simulink model "HFMA_4B_1_5_9_13"  (R2026b)
settings: Solver=FixedStepDiscrete  StopTime=stopTime  FixedStep=Ts
PreLoadFcn:
  | load('a_luts.mat')
values from neighbouring files (symbols this model uses):
  cosLUT = [1 1 1 1 1 1 1 1 1 1 1 1 ... (640 elements, 16x40)]    [iq_luts.mat]
  k_avg = 10    [Simulink_DOA_Test.m]    (also in collect_ranges.m; optimised_error_code.m)
  sinLUT = [0 0 0 0 0 0 0 0 0 0 0 0 ... (640 elements, 16x40)]    [iq_luts.mat]
  Ts = 1/8000    (= 0.000125)    [Simulink_DOA_Test.m]    (also in collect_ranges.m; optimised_error_code.m)
undefined symbols (not defined in the file or in its folder): a2_Im, a2_Re, a3_Im, a3_Re, NumBits1, NumBits2, Slope1, Slope2
libraries: hdlsllib x4, sl_signal_attributes x2
(part 5 of 6)

== system HFMA_4B_1_5_9_13/Subsystem/HFMA9/I//Q Separation2 ==
  note: -2x[n]*sin((2*pi*f0*n)/fs)
  note: 2x[n]*cos((2*pi*f0*n)/fs)
  Microphone Input : Inport
  F0 Index : Inport  Port=2
  IQ Counter Input : Inport  Port=3
  Gain : Gain  Gain=-2  ParamDataTypeStr=fixdt(1,18,16)  OutDataTypeStr=fixdt(1,18,14)  SaturateOnIntegerOverflow=on
  Gain1 : Gain  Gain=2  ParamDataTypeStr=fixdt(0,18,16)  OutDataTypeStr=fixdt(1,18,14)  SaturateOnIntegerOverflow=on
  IdxConv{,1..3} (4 alike) : DataTypeConversion  OutDataTypeStr=uint8  RndMeth=Floor
  Product : Product  OutDataTypeStr=fixdt(1,18,15)  SaturateOnIntegerOverflow=on
  Product1 : Product  OutDataTypeStr=fixdt(1,18,15)  SaturateOnIntegerOverflow=on
  cosLUT : LookupNDDirect  Table=[cosLUT]  TableDataTypeStr=fixdt(1,18,16)
  sinLUT : LookupNDDirect  Table=[sinLUT]  TableDataTypeStr=fixdt(1,18,16)
  I[n] : Outport
  Q[n] : Outport  Port=2
  wires:
  Gain/1 -> Q[n]/1
  Gain1/1 -> I[n]/1
  Microphone Input/1 -> Product1/1, Product/1
  cosLUT/1 -> Product/2
  sinLUT/1 -> Product1/2
  Product/1 -> Gain1/1
  Product1/1 -> Gain/1
  F0 Index/1 -> IdxConv/1, IdxConv2/1
  IQ Counter Input/1 -> IdxConv1/1, IdxConv3/1
  IdxConv/1 -> cosLUT/1
  IdxConv1/1 -> cosLUT/2
  IdxConv2/1 -> sinLUT/1
  IdxConv3/1 -> sinLUT/2

== system HFMA_4B_1_5_9_13/Subsystem/HFMA9/I//Q Separation3 ==
  note: -2x[n]*sin((2*pi*f0*n)/fs)
  note: 2x[n]*cos((2*pi*f0*n)/fs)
  Microphone Input : Inport
  F0 Index : Inport  Port=2
  IQ Counter Input : Inport  Port=3
  Gain : Gain  Gain=-2  ParamDataTypeStr=fixdt(1,18,16)  OutDataTypeStr=fixdt(1,18,14)  SaturateOnIntegerOverflow=on
  Gain1 : Gain  Gain=2  ParamDataTypeStr=fixdt(0,18,16)  OutDataTypeStr=fixdt(1,18,14)  SaturateOnIntegerOverflow=on
  IdxConv{,1..3} (4 alike) : DataTypeConversion  OutDataTypeStr=uint8  RndMeth=Floor
  Product : Product  OutDataTypeStr=fixdt(1,18,15)  SaturateOnIntegerOverflow=on
  Product1 : Product  OutDataTypeStr=fixdt(1,18,15)  SaturateOnIntegerOverflow=on
  cosLUT : LookupNDDirect  Table=[cosLUT]  TableDataTypeStr=fixdt(1,18,16)
  sinLUT : LookupNDDirect  Table=[sinLUT]  TableDataTypeStr=fixdt(1,18,16)
  I[n] : Outport
  Q[n] : Outport  Port=2
  wires:
  Gain/1 -> Q[n]/1
  Gain1/1 -> I[n]/1
  Microphone Input/1 -> Product1/1, Product/1
  cosLUT/1 -> Product/2
  sinLUT/1 -> Product1/2
  Product/1 -> Gain1/1
  Product1/1 -> Gain/1
  F0 Index/1 -> IdxConv/1, IdxConv2/1
  IQ Counter Input/1 -> IdxConv1/1, IdxConv3/1
  IdxConv/1 -> cosLUT/1
  IdxConv1/1 -> cosLUT/2
  IdxConv2/1 -> sinLUT/1
  IdxConv3/1 -> sinLUT/2

== system HFMA_4B_1_5_9_13/Subsystem/Max Theta Selector/Compare To Constant ==
  u : Inport
  Compare : RelationalOperator  Operator=<=  OutDataTypeStr=boolean
  Constant : Constant  DisableCoverage=on  Value=const  OutDataTypeStr=Inherit: Inherit via back propagation  SampleTime=-1
  y : Outport
  wires:
  Compare/1 -> y/1
  Constant/1 -> Compare/2
  u/1 -> Compare/1

== system HFMA_4B_1_5_9_13/Subsystem/Max Theta Selector/Compare To Constant1 ==
  u : Inport
  Compare : RelationalOperator  Operator===  OutDataTypeStr=boolean
  Constant : Constant  DisableCoverage=on  Value=const  OutDataTypeStr=Inherit: Inherit via back propagation  SampleTime=-1
  y : Outport
  wires:
  Compare/1 -> y/1
  Constant/1 -> Compare/2
  u/1 -> Compare/1

== system HFMA_4B_1_5_9_13/Subsystem/HFMA1/Covariance Matrix/R1 ==
  Xi_Re : Inport
  Xi_Im : Inport  Port=2
  Xj_Re : Inport  Port=3
  Xj_Im : Inport  Port=4
  RESET : Inport  Port=5
  Leaky Average : Subsystem
  Leaky Average1 : Subsystem
  ac_bd : Subsystem
  bc_ad : Subsystem
  Rij_Re : Outport
  Rij_Im : Outport  Port=2
  wires:
  Xi_Im/1 -> bc_ad/2(In2), ac_bd/2(In2)
  Xj_Im/1 -> bc_ad/4(In4), ac_bd/4(In4)
  Xj_Re/1 -> bc_ad/3(In3), ac_bd/3(In3)
  Xi_Re/1 -> bc_ad/1(In1), ac_bd/1(In1)
  ac_bd/1(Out1) -> Leaky Average/1(p[n])
  bc_ad/1(Out1) -> Leaky Average1/1(p[n])
  Leaky Average/1(Rij Out) -> Rij_Re/1
  RESET/1 -> Leaky Average1/2(RESET), Leaky Average/2(RESET)
  Leaky Average1/1(Rij Out) -> Rij_Im/1

== system HFMA_4B_1_5_9_13/Subsystem/HFMA1/Covariance Matrix/R2 ==
  Xi_Re : Inport
  Xi_Im : Inport  Port=2
  Xj_Re : Inport  Port=3
  Xj_Im : Inport  Port=4
  RESET : Inport  Port=5
  Leaky Average : Subsystem
  Leaky Average1 : Subsystem
  ac_bd : Subsystem
  bc_ad : Subsystem
  Rij_Re : Outport
  Rij_Im : Outport  Port=2
  wires:
  Xi_Im/1 -> bc_ad/2(In2), ac_bd/2(In2)
  Xj_Im/1 -> bc_ad/4(In4), ac_bd/4(In4)
  Xj_Re/1 -> bc_ad/3(In3), ac_bd/3(In3)
  Xi_Re/1 -> bc_ad/1(In1), ac_bd/1(In1)
  ac_bd/1(Out1) -> Leaky Average/1(p[n])
  bc_ad/1(Out1) -> Leaky Average1/1(p[n])
  Leaky Average/1(Rij Out) -> Rij_Re/1
  RESET/1 -> Leaky Average1/2(RESET), Leaky Average/2(RESET)
  Leaky Average1/1(Rij Out) -> Rij_Im/1

== system HFMA_4B_1_5_9_13/Subsystem/HFMA1/Covariance Matrix/R21 ==
  Xi_Re : Inport
  Xi_Im : Inport  Port=2
  Xj_Re : Inport  Port=3
  Xj_Im : Inport  Port=4
  RESET : Inport  Port=5
  Leaky Average : Subsystem
  Leaky Average1 : Subsystem
  ac_bd : Subsystem
  bc_ad : Subsystem
  Rij_Re : Outport
  Rij_Im : Outport  Port=2
  wires:
  Xi_Im/1 -> bc_ad/2(In2), ac_bd/2(In2)
  Xj_Im/1 -> bc_ad/4(In4), ac_bd/4(In4)
  Xj_Re/1 -> bc_ad/3(In3), ac_bd/3(In3)
  Xi_Re/1 -> bc_ad/1(In1), ac_bd/1(In1)
  ac_bd/1(Out1) -> Leaky Average/1(p[n])
  bc_ad/1(Out1) -> Leaky Average1/1(p[n])
  Leaky Average/1(Rij Out) -> Rij_Re/1
  RESET/1 -> Leaky Average1/2(RESET), Leaky Average/2(RESET)
  Leaky Average1/1(Rij Out) -> Rij_Im/1

== system HFMA_4B_1_5_9_13/Subsystem/HFMA1/Hardware Friendly MUSIC Algorithm/complex multiplier1 ==
  note: Rij'*an = (xu - yv) + j(xv+yu)
  x : Inport
  y : Inport  Port=2
  u : Inport  Port=3
  v : Inport  Port=4
  Add : Sum  Inputs=+-  OutDataTypeStr=fixdt(1,32,29)  SaturateOnIntegerOverflow=on
  Add1 : Sum  OutDataTypeStr=fixdt(1,32,29)  SaturateOnIntegerOverflow=on
  Product{,1..3} (4 alike) : Product  OutDataTypeStr=fixdt(1,32,29)  SaturateOnIntegerOverflow=on
  Re : Outport
  Im : Outport  Port=2
  wires:
  x/1 -> Product2/1, Product/1
  u/1 -> Product3/2, Product/2
  y/1 -> Product3/1, Product1/1
  v/1 -> Product2/2, Product1/2
  Product/1 -> Add/1
  Product1/1 -> Add/2
  Product2/1 -> Add1/1
  Product3/1 -> Add1/2
  Add/1 -> Re/1
  Add1/1 -> Im/1

== system HFMA_4B_1_5_9_13/Subsystem/HFMA1/Hardware Friendly MUSIC Algorithm/complex multiplier2 ==
  note: Rij'*an = (xu - yv) + j(xv+yu)
  x : Inport
  y : Inport  Port=2
  u : Inport  Port=3
  v : Inport  Port=4
  Add : Sum  Inputs=+-  OutDataTypeStr=fixdt(1,32,29)  SaturateOnIntegerOverflow=on
  Add1 : Sum  OutDataTypeStr=fixdt(1,32,29)  SaturateOnIntegerOverflow=on
  Product{,1..3} (4 alike) : Product  OutDataTypeStr=fixdt(1,32,29)  SaturateOnIntegerOverflow=on
  Re : Outport
  Im : Outport  Port=2
  wires:
  x/1 -> Product2/1, Product/1
  u/1 -> Product3/2, Product/2
  y/1 -> Product3/1, Product1/1
  v/1 -> Product2/2, Product1/2
  Product/1 -> Add/1
  Product1/1 -> Add/2
  Product2/1 -> Add1/1
  Product3/1 -> Add1/2
  Add/1 -> Re/1
  Add1/1 -> Im/1

== system HFMA_4B_1_5_9_13/Subsystem/HFMA1/Hardware Friendly MUSIC Algorithm/complex multiplier3 ==
  note: Rij'*an = (xu - yv) + j(xv+yu)
  x : Inport
  y : Inport  Port=2
  u : Inport  Port=3
  v : Inport  Port=4
  Add : Sum  Inputs=+-  OutDataTypeStr=fixdt(1,32,29)  SaturateOnIntegerOverflow=on
  Add1 : Sum  OutDataTypeStr=fixdt(1,32,29)  SaturateOnIntegerOverflow=on
  Product{,1..3} (4 alike) : Product  OutDataTypeStr=fixdt(1,32,29)  SaturateOnIntegerOverflow=on
  Re : Outport
  Im : Outport  Port=2
  wires:
  x/1 -> Product2/1, Product/1
  u/1 -> Product3/2, Product/2
  y/1 -> Product3/1, Product1/1
  v/1 -> Product2/2, Product1/2
  Product/1 -> Add/1
  Product1/1 -> Add/2
  Product2/1 -> Add1/1
  Product3/1 -> Add1/2
  Add/1 -> Re/1
  Add1/1 -> Im/1

== system HFMA_4B_1_5_9_13/Subsystem/HFMA13/Covariance Matrix/R1 ==
  Xi_Re : Inport
  Xi_Im : Inport  Port=2
  Xj_Re : Inport  Port=3
  Xj_Im : Inport  Port=4
  RESET : Inport  Port=5
  Leaky Average : Subsystem
  Leaky Average1 : Subsystem
  ac_bd : Subsystem
  bc_ad : Subsystem
  Rij_Re : Outport
  Rij_Im : Outport  Port=2
  wires:
  Xi_Im/1 -> bc_ad/2(In2), ac_bd/2(In2)
  Xj_Im/1 -> bc_ad/4(In4), ac_bd/4(In4)
  Xj_Re/1 -> bc_ad/3(In3), ac_bd/3(In3)
  Xi_Re/1 -> bc_ad/1(In1), ac_bd/1(In1)
  ac_bd/1(Out1) -> Leaky Average/1(p[n])
  bc_ad/1(Out1) -> Leaky Average1/1(p[n])
  Leaky Average/1(Rij Out) -> Rij_Re/1
  RESET/1 -> Leaky Average1/2(RESET), Leaky Average/2(RESET)
  Leaky Average1/1(Rij Out) -> Rij_Im/1

== system HFMA_4B_1_5_9_13/Subsystem/HFMA13/Covariance Matrix/R2 ==
  Xi_Re : Inport
  Xi_Im : Inport  Port=2
  Xj_Re : Inport  Port=3
  Xj_Im : Inport  Port=4
  RESET : Inport  Port=5
  Leaky Average : Subsystem
  Leaky Average1 : Subsystem
  ac_bd : Subsystem
  bc_ad : Subsystem
  Rij_Re : Outport
  Rij_Im : Outport  Port=2
  wires:
  Xi_Im/1 -> bc_ad/2(In2), ac_bd/2(In2)
  Xj_Im/1 -> bc_ad/4(In4), ac_bd/4(In4)
  Xj_Re/1 -> bc_ad/3(In3), ac_bd/3(In3)
  Xi_Re/1 -> bc_ad/1(In1), ac_bd/1(In1)
  ac_bd/1(Out1) -> Leaky Average/1(p[n])
  bc_ad/1(Out1) -> Leaky Average1/1(p[n])
  Leaky Average/1(Rij Out) -> Rij_Re/1
  RESET/1 -> Leaky Average1/2(RESET), Leaky Average/2(RESET)
  Leaky Average1/1(Rij Out) -> Rij_Im/1

== system HFMA_4B_1_5_9_13/Subsystem/HFMA13/Covariance Matrix/R21 ==
  Xi_Re : Inport
  Xi_Im : Inport  Port=2
  Xj_Re : Inport  Port=3
  Xj_Im : Inport  Port=4
  RESET : Inport  Port=5
  Leaky Average : Subsystem
  Leaky Average1 : Subsystem
  ac_bd : Subsystem
  bc_ad : Subsystem
  Rij_Re : Outport
  Rij_Im : Outport  Port=2
  wires:
  Xi_Im/1 -> bc_ad/2(In2), ac_bd/2(In2)
  Xj_Im/1 -> bc_ad/4(In4), ac_bd/4(In4)
  Xj_Re/1 -> bc_ad/3(In3), ac_bd/3(In3)
  Xi_Re/1 -> bc_ad/1(In1), ac_bd/1(In1)
  ac_bd/1(Out1) -> Leaky Average/1(p[n])
  bc_ad/1(Out1) -> Leaky Average1/1(p[n])
  Leaky Average/1(Rij Out) -> Rij_Re/1
  RESET/1 -> Leaky Average1/2(RESET), Leaky Average/2(RESET)
  Leaky Average1/1(Rij Out) -> Rij_Im/1

== system HFMA_4B_1_5_9_13/Subsystem/HFMA13/Hardware Friendly MUSIC Algorithm/complex multiplier1 ==
  note: Rij'*an = (xu - yv) + j(xv+yu)
  x : Inport
  y : Inport  Port=2
  u : Inport  Port=3
  v : Inport  Port=4
  Add : Sum  Inputs=+-  OutDataTypeStr=fixdt(1,32,29)  SaturateOnIntegerOverflow=on
  Add1 : Sum  OutDataTypeStr=fixdt(1,32,29)  SaturateOnIntegerOverflow=on
  Product{,1..3} (4 alike) : Product  OutDataTypeStr=fixdt(1,32,29)  SaturateOnIntegerOverflow=on
  Re : Outport
  Im : Outport  Port=2
  wires:
  x/1 -> Product2/1, Product/1
  u/1 -> Product3/2, Product/2
  y/1 -> Product3/1, Product1/1
  v/1 -> Product2/2, Product1/2
  Product/1 -> Add/1
  Product1/1 -> Add/2
  Product2/1 -> Add1/1
  Product3/1 -> Add1/2
  Add/1 -> Re/1
  Add1/1 -> Im/1

== system HFMA_4B_1_5_9_13/Subsystem/HFMA13/Hardware Friendly MUSIC Algorithm/complex multiplier2 ==
  note: Rij'*an = (xu - yv) + j(xv+yu)
  x : Inport
  y : Inport  Port=2
  u : Inport  Port=3
  v : Inport  Port=4
  Add : Sum  Inputs=+-  OutDataTypeStr=fixdt(1,32,29)  SaturateOnIntegerOverflow=on
  Add1 : Sum  OutDataTypeStr=fixdt(1,32,29)  SaturateOnIntegerOverflow=on
  Product{,1..3} (4 alike) : Product  OutDataTypeStr=fixdt(1,32,29)  SaturateOnIntegerOverflow=on
  Re : Outport
  Im : Outport  Port=2
  wires:
  x/1 -> Product2/1, Product/1
  u/1 -> Product3/2, Product/2
  y/1 -> Product3/1, Product1/1
  v/1 -> Product2/2, Product1/2
  Product/1 -> Add/1
  Product1/1 -> Add/2
  Product2/1 -> Add1/1
  Product3/1 -> Add1/2
  Add/1 -> Re/1
  Add1/1 -> Im/1

== system HFMA_4B_1_5_9_13/Subsystem/HFMA13/Hardware Friendly MUSIC Algorithm/complex multiplier3 ==
  note: Rij'*an = (xu - yv) + j(xv+yu)
  x : Inport
  y : Inport  Port=2
  u : Inport  Port=3
  v : Inport  Port=4
  Add : Sum  Inputs=+-  OutDataTypeStr=fixdt(1,32,29)  SaturateOnIntegerOverflow=on
  Add1 : Sum  OutDataTypeStr=fixdt(1,32,29)  SaturateOnIntegerOverflow=on
  Product{,1..3} (4 alike) : Product  OutDataTypeStr=fixdt(1,32,29)  SaturateOnIntegerOverflow=on
  Re : Outport
  Im : Outport  Port=2
  wires:
  x/1 -> Product2/1, Product/1
  u/1 -> Product3/2, Product/2
  y/1 -> Product3/1, Product1/1
  v/1 -> Product2/2, Product1/2
  Product/1 -> Add/1
  Product1/1 -> Add/2
  Product2/1 -> Add1/1
  Product3/1 -> Add1/2
  Add/1 -> Re/1
  Add1/1 -> Im/1

== system HFMA_4B_1_5_9_13/Subsystem/HFMA5/Covariance Matrix/R1 ==
  Xi_Re : Inport
  Xi_Im : Inport  Port=2
  Xj_Re : Inport  Port=3
  Xj_Im : Inport  Port=4
  RESET : Inport  Port=5
  Leaky Average : Subsystem
  Leaky Average1 : Subsystem
  ac_bd : Subsystem
  bc_ad : Subsystem
  Rij_Re : Outport
  Rij_Im : Outport  Port=2
  wires:
  Xi_Im/1 -> bc_ad/2(In2), ac_bd/2(In2)
  Xj_Im/1 -> bc_ad/4(In4), ac_bd/4(In4)
  Xj_Re/1 -> bc_ad/3(In3), ac_bd/3(In3)
  Xi_Re/1 -> bc_ad/1(In1), ac_bd/1(In1)
  ac_bd/1(Out1) -> Leaky Average/1(p[n])
  bc_ad/1(Out1) -> Leaky Average1/1(p[n])
  Leaky Average/1(Rij Out) -> Rij_Re/1
  RESET/1 -> Leaky Average1/2(RESET), Leaky Average/2(RESET)
  Leaky Average1/1(Rij Out) -> Rij_Im/1

== system HFMA_4B_1_5_9_13/Subsystem/HFMA5/Covariance Matrix/R2 ==
  Xi_Re : Inport
  Xi_Im : Inport  Port=2
  Xj_Re : Inport  Port=3
  Xj_Im : Inport  Port=4
  RESET : Inport  Port=5
  Leaky Average : Subsystem
  Leaky Average1 : Subsystem
  ac_bd : Subsystem
  bc_ad : Subsystem
  Rij_Re : Outport
  Rij_Im : Outport  Port=2
  wires:
  Xi_Im/1 -> bc_ad/2(In2), ac_bd/2(In2)
  Xj_Im/1 -> bc_ad/4(In4), ac_bd/4(In4)
  Xj_Re/1 -> bc_ad/3(In3), ac_bd/3(In3)
  Xi_Re/1 -> bc_ad/1(In1), ac_bd/1(In1)
  ac_bd/1(Out1) -> Leaky Average/1(p[n])
  bc_ad/1(Out1) -> Leaky Average1/1(p[n])
  Leaky Average/1(Rij Out) -> Rij_Re/1
  RESET/1 -> Leaky Average1/2(RESET), Leaky Average/2(RESET)
  Leaky Average1/1(Rij Out) -> Rij_Im/1

== system HFMA_4B_1_5_9_13/Subsystem/HFMA5/Covariance Matrix/R21 ==
  Xi_Re : Inport
  Xi_Im : Inport  Port=2
  Xj_Re : Inport  Port=3
  Xj_Im : Inport  Port=4
  RESET : Inport  Port=5
  Leaky Average : Subsystem
  Leaky Average1 : Subsystem
  ac_bd : Subsystem
  bc_ad : Subsystem
  Rij_Re : Outport
  Rij_Im : Outport  Port=2
  wires:
  Xi_Im/1 -> bc_ad/2(In2), ac_bd/2(In2)
  Xj_Im/1 -> bc_ad/4(In4), ac_bd/4(In4)
  Xj_Re/1 -> bc_ad/3(In3), ac_bd/3(In3)
  Xi_Re/1 -> bc_ad/1(In1), ac_bd/1(In1)
  ac_bd/1(Out1) -> Leaky Average/1(p[n])
  bc_ad/1(Out1) -> Leaky Average1/1(p[n])
  Leaky Average/1(Rij Out) -> Rij_Re/1
  RESET/1 -> Leaky Average1/2(RESET), Leaky Average/2(RESET)
  Leaky Average1/1(Rij Out) -> Rij_Im/1

== system HFMA_4B_1_5_9_13/Subsystem/HFMA5/Hardware Friendly MUSIC Algorithm/complex multiplier1 ==
  note: Rij'*an = (xu - yv) + j(xv+yu)
  x : Inport
  y : Inport  Port=2
  u : Inport  Port=3
  v : Inport  Port=4
  Add : Sum  Inputs=+-  OutDataTypeStr=fixdt(1,32,29)  SaturateOnIntegerOverflow=on
  Add1 : Sum  OutDataTypeStr=fixdt(1,32,29)  SaturateOnIntegerOverflow=on
  Product{,1..3} (4 alike) : Product  OutDataTypeStr=fixdt(1,32,29)  SaturateOnIntegerOverflow=on
  Re : Outport
  Im : Outport  Port=2
  wires:
  x/1 -> Product2/1, Product/1
  u/1 -> Product3/2, Product/2
  y/1 -> Product3/1, Product1/1
  v/1 -> Product2/2, Product1/2
  Product/1 -> Add/1
  Product1/1 -> Add/2
  Product2/1 -> Add1/1
  Product3/1 -> Add1/2
  Add/1 -> Re/1
  Add1/1 -> Im/1

== system HFMA_4B_1_5_9_13/Subsystem/HFMA5/Hardware Friendly MUSIC Algorithm/complex multiplier2 ==
  note: Rij'*an = (xu - yv) + j(xv+yu)
  x : Inport
  y : Inport  Port=2
  u : Inport  Port=3
  v : Inport  Port=4
  Add : Sum  Inputs=+-  OutDataTypeStr=fixdt(1,32,29)  SaturateOnIntegerOverflow=on
  Add1 : Sum  OutDataTypeStr=fixdt(1,32,29)  SaturateOnIntegerOverflow=on
  Product{,1..3} (4 alike) : Product  OutDataTypeStr=fixdt(1,32,29)  SaturateOnIntegerOverflow=on
  Re : Outport
  Im : Outport  Port=2
  wires:
  x/1 -> Product2/1, Product/1
  u/1 -> Product3/2, Product/2
  y/1 -> Product3/1, Product1/1
  v/1 -> Product2/2, Product1/2
  Product/1 -> Add/1
  Product1/1 -> Add/2
  Product2/1 -> Add1/1
  Product3/1 -> Add1/2
  Add/1 -> Re/1
  Add1/1 -> Im/1

== system HFMA_4B_1_5_9_13/Subsystem/HFMA5/Hardware Friendly MUSIC Algorithm/complex multiplier3 ==
  note: Rij'*an = (xu - yv) + j(xv+yu)
  x : Inport
  y : Inport  Port=2
  u : Inport  Port=3
  v : Inport  Port=4
  Add : Sum  Inputs=+-  OutDataTypeStr=fixdt(1,32,29)  SaturateOnIntegerOverflow=on
  Add1 : Sum  OutDataTypeStr=fixdt(1,32,29)  SaturateOnIntegerOverflow=on
  Product{,1..3} (4 alike) : Product  OutDataTypeStr=fixdt(1,32,29)  SaturateOnIntegerOverflow=on
  Re : Outport
  Im : Outport  Port=2
  wires:
  x/1 -> Product2/1, Product/1
  u/1 -> Product3/2, Product/2
  y/1 -> Product3/1, Product1/1
  v/1 -> Product2/2, Product1/2
  Product/1 -> Add/1
  Product1/1 -> Add/2
  Product2/1 -> Add1/1
  Product3/1 -> Add1/2
  Add/1 -> Re/1
  Add1/1 -> Im/1

== system HFMA_4B_1_5_9_13/Subsystem/HFMA9/Covariance Matrix/R1 ==
  Xi_Re : Inport
  Xi_Im : Inport  Port=2
  Xj_Re : Inport  Port=3
  Xj_Im : Inport  Port=4
  RESET : Inport  Port=5
  Leaky Average : Subsystem
  Leaky Average1 : Subsystem
  ac_bd : Subsystem
  bc_ad : Subsystem
  Rij_Re : Outport
  Rij_Im : Outport  Port=2
  wires:
  Xi_Im/1 -> bc_ad/2(In2), ac_bd/2(In2)
  Xj_Im/1 -> bc_ad/4(In4), ac_bd/4(In4)
  Xj_Re/1 -> bc_ad/3(In3), ac_bd/3(In3)
  Xi_Re/1 -> bc_ad/1(In1), ac_bd/1(In1)
  ac_bd/1(Out1) -> Leaky Average/1(p[n])
  bc_ad/1(Out1) -> Leaky Average1/1(p[n])
  Leaky Average/1(Rij Out) -> Rij_Re/1
  RESET/1 -> Leaky Average1/2(RESET), Leaky Average/2(RESET)
  Leaky Average1/1(Rij Out) -> Rij_Im/1

== system HFMA_4B_1_5_9_13/Subsystem/HFMA9/Covariance Matrix/R2 ==
  Xi_Re : Inport
  Xi_Im : Inport  Port=2
  Xj_Re : Inport  Port=3
  Xj_Im : Inport  Port=4
  RESET : Inport  Port=5
  Leaky Average : Subsystem
  Leaky Average1 : Subsystem
  ac_bd : Subsystem
  bc_ad : Subsystem
  Rij_Re : Outport
  Rij_Im : Outport  Port=2
  wires:
  Xi_Im/1 -> bc_ad/2(In2), ac_bd/2(In2)
  Xj_Im/1 -> bc_ad/4(In4), ac_bd/4(In4)
  Xj_Re/1 -> bc_ad/3(In3), ac_bd/3(In3)
  Xi_Re/1 -> bc_ad/1(In1), ac_bd/1(In1)
  ac_bd/1(Out1) -> Leaky Average/1(p[n])
  bc_ad/1(Out1) -> Leaky Average1/1(p[n])
  Leaky Average/1(Rij Out) -> Rij_Re/1
  RESET/1 -> Leaky Average1/2(RESET), Leaky Average/2(RESET)
  Leaky Average1/1(Rij Out) -> Rij_Im/1

== system HFMA_4B_1_5_9_13/Subsystem/HFMA9/Covariance Matrix/R21 ==
  Xi_Re : Inport
  Xi_Im : Inport  Port=2
  Xj_Re : Inport  Port=3
  Xj_Im : Inport  Port=4
  RESET : Inport  Port=5
  Leaky Average : Subsystem
  Leaky Average1 : Subsystem
  ac_bd : Subsystem
  bc_ad : Subsystem
  Rij_Re : Outport
  Rij_Im : Outport  Port=2
  wires:
  Xi_Im/1 -> bc_ad/2(In2), ac_bd/2(In2)
  Xj_Im/1 -> bc_ad/4(In4), ac_bd/4(In4)
  Xj_Re/1 -> bc_ad/3(In3), ac_bd/3(In3)
  Xi_Re/1 -> bc_ad/1(In1), ac_bd/1(In1)
  ac_bd/1(Out1) -> Leaky Average/1(p[n])
  bc_ad/1(Out1) -> Leaky Average1/1(p[n])
  Leaky Average/1(Rij Out) -> Rij_Re/1
  RESET/1 -> Leaky Average1/2(RESET), Leaky Average/2(RESET)
  Leaky Average1/1(Rij Out) -> Rij_Im/1

== system HFMA_4B_1_5_9_13/Subsystem/HFMA9/Hardware Friendly MUSIC Algorithm/complex multiplier1 ==
  note: Rij'*an = (xu - yv) + j(xv+yu)
  x : Inport
  y : Inport  Port=2
  u : Inport  Port=3
  v : Inport  Port=4
  Add : Sum  Inputs=+-  OutDataTypeStr=fixdt(1,32,29)  SaturateOnIntegerOverflow=on
  Add1 : Sum  OutDataTypeStr=fixdt(1,32,29)  SaturateOnIntegerOverflow=on
  Product{,1..3} (4 alike) : Product  OutDataTypeStr=fixdt(1,32,29)  SaturateOnIntegerOverflow=on
  Re : Outport
  Im : Outport  Port=2
  wires:
  x/1 -> Product2/1, Product/1
  u/1 -> Product3/2, Product/2
  y/1 -> Product3/1, Product1/1
  v/1 -> Product2/2, Product1/2
  Product/1 -> Add/1
  Product1/1 -> Add/2
  Product2/1 -> Add1/1
  Product3/1 -> Add1/2
  Add/1 -> Re/1
  Add1/1 -> Im/1

== system HFMA_4B_1_5_9_13/Subsystem/HFMA9/Hardware Friendly MUSIC Algorithm/complex multiplier2 ==
  note: Rij'*an = (xu - yv) + j(xv+yu)
  x : Inport
  y : Inport  Port=2
  u : Inport  Port=3
  v : Inport  Port=4
  Add : Sum  Inputs=+-  OutDataTypeStr=fixdt(1,32,29)  SaturateOnIntegerOverflow=on
  Add1 : Sum  OutDataTypeStr=fixdt(1,32,29)  SaturateOnIntegerOverflow=on
  Product{,1..3} (4 alike) : Product  OutDataTypeStr=fixdt(1,32,29)  SaturateOnIntegerOverflow=on
  Re : Outport
  Im : Outport  Port=2
  wires:
  x/1 -> Product2/1, Product/1
  u/1 -> Product3/2, Product/2
  y/1 -> Product3/1, Product1/1
  v/1 -> Product2/2, Product1/2
  Product/1 -> Add/1
  Product1/1 -> Add/2
  Product2/1 -> Add1/1
  Product3/1 -> Add1/2
  Add/1 -> Re/1
  Add1/1 -> Im/1

== system HFMA_4B_1_5_9_13/Subsystem/HFMA9/Hardware Friendly MUSIC Algorithm/complex multiplier3 ==
  note: Rij'*an = (xu - yv) + j(xv+yu)
  x : Inport
  y : Inport  Port=2
  u : Inport  Port=3
  v : Inport  Port=4
  Add : Sum  Inputs=+-  OutDataTypeStr=fixdt(1,32,29)  SaturateOnIntegerOverflow=on
  Add1 : Sum  OutDataTypeStr=fixdt(1,32,29)  SaturateOnIntegerOverflow=on
  Product{,1..3} (4 alike) : Product  OutDataTypeStr=fixdt(1,32,29)  SaturateOnIntegerOverflow=on
  Re : Outport
  Im : Outport  Port=2
  wires:
  x/1 -> Product2/1, Product/1
  u/1 -> Product3/2, Product/2
  y/1 -> Product3/1, Product1/1
  v/1 -> Product2/2, Product1/2
  Product/1 -> Add/1
  Product1/1 -> Add/2
  Product2/1 -> Add1/1
  Product3/1 -> Add1/2
  Add/1 -> Re/1
  Add1/1 -> Im/1

== system HFMA_4B_1_5_9_13/Subsystem/HFMA1/Covariance Matrix/R1/Leaky Average ==
  p[n] : Inport
  RESET : Inport  Port=2
  Add : Sum  OutDataTypeStr=fixdt(1,32,30)  SaturateOnIntegerOverflow=on
  Delay : Delay  DelayLength=1  ExternalReset=Level
      settings: InputPortMap=u0,r5
  Gain : Gain  Gain=2^-k_avg  OutDataTypeStr=fixdt(1,32,30)  SaturateOnIntegerOverflow=on
  Minus : Sum  Inputs=+-  OutDataTypeStr=fixdt(1,32,30)  SaturateOnIntegerOverflow=on
  Rij Out : Outport
  wires:
  p[n]/1 -> Minus/1
  Minus/1 -> Gain/1
  Gain/1 -> Add/1
  Add/1 -> Delay/1
  Delay/1 -> Rij Out/1, Minus/2, Add/2
  RESET/1 -> Delay/2

== system HFMA_4B_1_5_9_13/Subsystem/HFMA1/Covariance Matrix/R1/Leaky Average1 ==
  p[n] : Inport
  RESET : Inport  Port=2
  Add : Sum  OutDataTypeStr=fixdt(1,32,30)  SaturateOnIntegerOverflow=on
  Delay : Delay  DelayLength=1  ExternalReset=Level
      settings: InputPortMap=u0,r5
  Gain : Gain  Gain=2^-k_avg  OutDataTypeStr=fixdt(1,32,30)  SaturateOnIntegerOverflow=on
  Minus : Sum  Inputs=+-  OutDataTypeStr=fixdt(1,32,30)  SaturateOnIntegerOverflow=on
  Rij Out : Outport
  wires:
  p[n]/1 -> Minus/1
  Minus/1 -> Gain/1
  Gain/1 -> Add/1
  Add/1 -> Delay/1
  Delay/1 -> Rij Out/1, Minus/2, Add/2
  RESET/1 -> Delay/2

== system HFMA_4B_1_5_9_13/Subsystem/HFMA1/Covariance Matrix/R1/ac_bd ==
  In1 : Inport
  In2 : Inport  Port=2
  In3 : Inport  Port=3
  In4 : Inport  Port=4
  Add : Sum  OutDataTypeStr=fixdt(1,32,30)  SaturateOnIntegerOverflow=on
  Product : Product  OutDataTypeStr=fixdt(1,32,30)  SaturateOnIntegerOverflow=on
  Product1 : Product  OutDataTypeStr=fixdt(1,32,30)  SaturateOnIntegerOverflow=on
  Out1 : Outport
  wires:
  In1/1 -> Product/1
  In3/1 -> Product/2
  In2/1 -> Product1/1
  In4/1 -> Product1/2
  Product/1 -> Add/1
  Product1/1 -> Add/2
  Add/1 -> Out1/1

== system HFMA_4B_1_5_9_13/Subsystem/HFMA1/Covariance Matrix/R1/bc_ad ==
  In1 : Inport
  In2 : Inport  Port=2
  In3 : Inport  Port=3
  In4 : Inport  Port=4
  Product : Product  OutDataTypeStr=fixdt(1,32,30)  SaturateOnIntegerOverflow=on
  Product1 : Product  OutDataTypeStr=fixdt(1,32,30)  SaturateOnIntegerOverflow=on
  Subtract : Sum  Inputs=+-  OutDataTypeStr=fixdt(1,32,30)  SaturateOnIntegerOverflow=on
  Out1 : Outport
  wires:
  In2/1 -> Product/1
  In3/1 -> Product/2
  In1/1 -> Product1/1
  In4/1 -> Product1/2
  Product/1 -> Subtract/1
  Product1/1 -> Subtract/2
  Subtract/1 -> Out1/1

== system HFMA_4B_1_5_9_13/Subsystem/HFMA1/Covariance Matrix/R2/Leaky Average ==
  p[n] : Inport
  RESET : Inport  Port=2
  Add : Sum  OutDataTypeStr=fixdt(1,32,30)  SaturateOnIntegerOverflow=on
  Delay : Delay  DelayLength=1  ExternalReset=Level
      settings: InputPortMap=u0,r5
  Gain : Gain  Gain=2^-k_avg  OutDataTypeStr=fixdt(1,32,30)  SaturateOnIntegerOverflow=on
  Minus : Sum  Inputs=+-  OutDataTypeStr=fixdt(1,32,30)  SaturateOnIntegerOverflow=on
  Rij Out : Outport
  wires:
  p[n]/1 -> Minus/1
  Minus/1 -> Gain/1
  Gain/1 -> Add/1
  Add/1 -> Delay/1
  Delay/1 -> Rij Out/1, Minus/2, Add/2
  RESET/1 -> Delay/2

== system HFMA_4B_1_5_9_13/Subsystem/HFMA1/Covariance Matrix/R2/Leaky Average1 ==
  p[n] : Inport
  RESET : Inport  Port=2
  Add : Sum  OutDataTypeStr=fixdt(1,32,30)  SaturateOnIntegerOverflow=on
  Delay : Delay  DelayLength=1  ExternalReset=Level
      settings: InputPortMap=u0,r5
  Gain : Gain  Gain=2^-k_avg  OutDataTypeStr=fixdt(1,32,30)  SaturateOnIntegerOverflow=on
  Minus : Sum  Inputs=+-  OutDataTypeStr=fixdt(1,32,30)  SaturateOnIntegerOverflow=on
  Rij Out : Outport
  wires:
  p[n]/1 -> Minus/1
  Minus/1 -> Gain/1
  Gain/1 -> Add/1
  Add/1 -> Delay/1
  Delay/1 -> Rij Out/1, Minus/2, Add/2
  RESET/1 -> Delay/2

== system HFMA_4B_1_5_9_13/Subsystem/HFMA1/Covariance Matrix/R2/ac_bd ==
  In1 : Inport
  In2 : Inport  Port=2
  In3 : Inport  Port=3
  In4 : Inport  Port=4
  Add : Sum  OutDataTypeStr=fixdt(1,32,30)  SaturateOnIntegerOverflow=on
  Product : Product  OutDataTypeStr=fixdt(1,32,30)  SaturateOnIntegerOverflow=on
  Product1 : Product  OutDataTypeStr=fixdt(1,32,30)  SaturateOnIntegerOverflow=on
  Out1 : Outport
  wires:
  In1/1 -> Product/1
  In3/1 -> Product/2
  In2/1 -> Product1/1
  In4/1 -> Product1/2
  Product/1 -> Add/1
  Product1/1 -> Add/2
  Add/1 -> Out1/1

== system HFMA_4B_1_5_9_13/Subsystem/HFMA1/Covariance Matrix/R2/bc_ad ==
  In1 : Inport
  In2 : Inport  Port=2
  In3 : Inport  Port=3
  In4 : Inport  Port=4
  Product : Product  OutDataTypeStr=fixdt(1,32,30)  SaturateOnIntegerOverflow=on
  Product1 : Product  OutDataTypeStr=fixdt(1,32,30)  SaturateOnIntegerOverflow=on
  Subtract : Sum  Inputs=+-  OutDataTypeStr=fixdt(1,32,30)  SaturateOnIntegerOverflow=on
  Out1 : Outport
  wires:
  In2/1 -> Product/1
  In3/1 -> Product/2
  In1/1 -> Product1/1
  In4/1 -> Product1/2
  Product/1 -> Subtract/1
  Product1/1 -> Subtract/2
  Subtract/1 -> Out1/1

== system HFMA_4B_1_5_9_13/Subsystem/HFMA1/Covariance Matrix/R21/Leaky Average ==
  p[n] : Inport
  RESET : Inport  Port=2
  Add : Sum  OutDataTypeStr=fixdt(1,32,30)  SaturateOnIntegerOverflow=on
  Delay : Delay  DelayLength=1  ExternalReset=Level
      settings: InputPortMap=u0,r5
  Gain : Gain  Gain=2^-k_avg  OutDataTypeStr=fixdt(1,32,30)  SaturateOnIntegerOverflow=on
  Minus : Sum  Inputs=+-  OutDataTypeStr=fixdt(1,32,30)  SaturateOnIntegerOverflow=on
  Rij Out : Outport
  wires:
  p[n]/1 -> Minus/1
  Minus/1 -> Gain/1
  Gain/1 -> Add/1
  Add/1 -> Delay/1
  Delay/1 -> Rij Out/1, Minus/2, Add/2
  RESET/1 -> Delay/2

== system HFMA_4B_1_5_9_13/Subsystem/HFMA1/Covariance Matrix/R21/Leaky Average1 ==
  p[n] : Inport
  RESET : Inport  Port=2
  Add : Sum  OutDataTypeStr=fixdt(1,32,30)  SaturateOnIntegerOverflow=on
  Delay : Delay  DelayLength=1  ExternalReset=Level
      settings: InputPortMap=u0,r5
  Gain : Gain  Gain=2^-k_avg  OutDataTypeStr=fixdt(1,32,30)  SaturateOnIntegerOverflow=on
  Minus : Sum  Inputs=+-  OutDataTypeStr=fixdt(1,32,30)  SaturateOnIntegerOverflow=on
  Rij Out : Outport
  wires:
  p[n]/1 -> Minus/1
  Minus/1 -> Gain/1
  Gain/1 -> Add/1
  Add/1 -> Delay/1
  Delay/1 -> Rij Out/1, Minus/2, Add/2
  RESET/1 -> Delay/2

== system HFMA_4B_1_5_9_13/Subsystem/HFMA1/Covariance Matrix/R21/ac_bd ==
  In1 : Inport
  In2 : Inport  Port=2
  In3 : Inport  Port=3
  In4 : Inport  Port=4
  Add : Sum  OutDataTypeStr=fixdt(1,32,30)  SaturateOnIntegerOverflow=on
  Product : Product  OutDataTypeStr=fixdt(1,32,30)  SaturateOnIntegerOverflow=on
  Product1 : Product  OutDataTypeStr=fixdt(1,32,30)  SaturateOnIntegerOverflow=on
  Out1 : Outport
  wires:
  In1/1 -> Product/1
  In3/1 -> Product/2
  In2/1 -> Product1/1
  In4/1 -> Product1/2
  Product/1 -> Add/1
  Product1/1 -> Add/2
  Add/1 -> Out1/1

== system HFMA_4B_1_5_9_13/Subsystem/HFMA1/Covariance Matrix/R21/bc_ad ==
  In1 : Inport
  In2 : Inport  Port=2
  In3 : Inport  Port=3
  In4 : Inport  Port=4
  Product : Product  OutDataTypeStr=fixdt(1,32,30)  SaturateOnIntegerOverflow=on
  Product1 : Product  OutDataTypeStr=fixdt(1,32,30)  SaturateOnIntegerOverflow=on
  Subtract : Sum  Inputs=+-  OutDataTypeStr=fixdt(1,32,30)  SaturateOnIntegerOverflow=on
  Out1 : Outport
  wires:
  In2/1 -> Product/1
  In3/1 -> Product/2
  In1/1 -> Product1/1
  In4/1 -> Product1/2
  Product/1 -> Subtract/1
  Product1/1 -> Subtract/2
  Subtract/1 -> Out1/1

== system HFMA_4B_1_5_9_13/Subsystem/HFMA13/Covariance Matrix/R1/Leaky Average ==
  p[n] : Inport
  RESET : Inport  Port=2
  Add : Sum  OutDataTypeStr=fixdt(1,32,30)  SaturateOnIntegerOverflow=on
  Delay : Delay  DelayLength=1  ExternalReset=Level
      settings: InputPortMap=u0,r5
  Gain : Gain  Gain=2^-k_avg  OutDataTypeStr=fixdt(1,32,30)  SaturateOnIntegerOverflow=on
  Minus : Sum  Inputs=+-  OutDataTypeStr=fixdt(1,32,30)  SaturateOnIntegerOverflow=on
  Rij Out : Outport
  wires:
  p[n]/1 -> Minus/1
  Minus/1 -> Gain/1
  Gain/1 -> Add/1
  Add/1 -> Delay/1
  Delay/1 -> Rij Out/1, Minus/2, Add/2
  RESET/1 -> Delay/2

== system HFMA_4B_1_5_9_13/Subsystem/HFMA13/Covariance Matrix/R1/Leaky Average1 ==
  p[n] : Inport
  RESET : Inport  Port=2
  Add : Sum  OutDataTypeStr=fixdt(1,32,30)  SaturateOnIntegerOverflow=on
  Delay : Delay  DelayLength=1  ExternalReset=Level
      settings: InputPortMap=u0,r5
  Gain : Gain  Gain=2^-k_avg  OutDataTypeStr=fixdt(1,32,30)  SaturateOnIntegerOverflow=on
  Minus : Sum  Inputs=+-  OutDataTypeStr=fixdt(1,32,30)  SaturateOnIntegerOverflow=on
  Rij Out : Outport
  wires:
  p[n]/1 -> Minus/1
  Minus/1 -> Gain/1
  Gain/1 -> Add/1
  Add/1 -> Delay/1
  Delay/1 -> Rij Out/1, Minus/2, Add/2
  RESET/1 -> Delay/2

== system HFMA_4B_1_5_9_13/Subsystem/HFMA13/Covariance Matrix/R1/ac_bd ==
  In1 : Inport
  In2 : Inport  Port=2
  In3 : Inport  Port=3
  In4 : Inport  Port=4
  Add : Sum  OutDataTypeStr=fixdt(1,32,30)  SaturateOnIntegerOverflow=on
  Product : Product  OutDataTypeStr=fixdt(1,32,30)  SaturateOnIntegerOverflow=on
  Product1 : Product  OutDataTypeStr=fixdt(1,32,30)  SaturateOnIntegerOverflow=on
  Out1 : Outport
  wires:
  In1/1 -> Product/1
  In3/1 -> Product/2
  In2/1 -> Product1/1
  In4/1 -> Product1/2
  Product/1 -> Add/1
  Product1/1 -> Add/2
  Add/1 -> Out1/1

== system HFMA_4B_1_5_9_13/Subsystem/HFMA13/Covariance Matrix/R1/bc_ad ==
  In1 : Inport
  In2 : Inport  Port=2
  In3 : Inport  Port=3
  In4 : Inport  Port=4
  Product : Product  OutDataTypeStr=fixdt(1,32,30)  SaturateOnIntegerOverflow=on
  Product1 : Product  OutDataTypeStr=fixdt(1,32,30)  SaturateOnIntegerOverflow=on
  Subtract : Sum  Inputs=+-  OutDataTypeStr=fixdt(1,32,30)  SaturateOnIntegerOverflow=on
  Out1 : Outport
  wires:
  In2/1 -> Product/1
  In3/1 -> Product/2
  In1/1 -> Product1/1
  In4/1 -> Product1/2
  Product/1 -> Subtract/1
  Product1/1 -> Subtract/2
  Subtract/1 -> Out1/1

== system HFMA_4B_1_5_9_13/Subsystem/HFMA13/Covariance Matrix/R2/Leaky Average ==
  p[n] : Inport
  RESET : Inport  Port=2
  Add : Sum  OutDataTypeStr=fixdt(1,32,30)  SaturateOnIntegerOverflow=on
  Delay : Delay  DelayLength=1  ExternalReset=Level
      settings: InputPortMap=u0,r5
  Gain : Gain  Gain=2^-k_avg  OutDataTypeStr=fixdt(1,32,30)  SaturateOnIntegerOverflow=on
  Minus : Sum  Inputs=+-  OutDataTypeStr=fixdt(1,32,30)  SaturateOnIntegerOverflow=on
  Rij Out : Outport
  wires:
  p[n]/1 -> Minus/1
  Minus/1 -> Gain/1
  Gain/1 -> Add/1
  Add/1 -> Delay/1
  Delay/1 -> Rij Out/1, Minus/2, Add/2
  RESET/1 -> Delay/2

== system HFMA_4B_1_5_9_13/Subsystem/HFMA13/Covariance Matrix/R2/Leaky Average1 ==
  p[n] : Inport
  RESET : Inport  Port=2
  Add : Sum  OutDataTypeStr=fixdt(1,32,30)  SaturateOnIntegerOverflow=on
  Delay : Delay  DelayLength=1  ExternalReset=Level
      settings: InputPortMap=u0,r5
  Gain : Gain  Gain=2^-k_avg  OutDataTypeStr=fixdt(1,32,30)  SaturateOnIntegerOverflow=on
  Minus : Sum  Inputs=+-  OutDataTypeStr=fixdt(1,32,30)  SaturateOnIntegerOverflow=on
  Rij Out : Outport
  wires:
  p[n]/1 -> Minus/1
  Minus/1 -> Gain/1
  Gain/1 -> Add/1
  Add/1 -> Delay/1
  Delay/1 -> Rij Out/1, Minus/2, Add/2
  RESET/1 -> Delay/2

== system HFMA_4B_1_5_9_13/Subsystem/HFMA13/Covariance Matrix/R2/ac_bd ==
  In1 : Inport
  In2 : Inport  Port=2
  In3 : Inport  Port=3
  In4 : Inport  Port=4
  Add : Sum  OutDataTypeStr=fixdt(1,32,30)  SaturateOnIntegerOverflow=on
  Product : Product  OutDataTypeStr=fixdt(1,32,30)  SaturateOnIntegerOverflow=on
  Product1 : Product  OutDataTypeStr=fixdt(1,32,30)  SaturateOnIntegerOverflow=on
  Out1 : Outport
  wires:
  In1/1 -> Product/1
  In3/1 -> Product/2
  In2/1 -> Product1/1
  In4/1 -> Product1/2
  Product/1 -> Add/1
  Product1/1 -> Add/2
  Add/1 -> Out1/1

== system HFMA_4B_1_5_9_13/Subsystem/HFMA13/Covariance Matrix/R2/bc_ad ==
  In1 : Inport
  In2 : Inport  Port=2
  In3 : Inport  Port=3
  In4 : Inport  Port=4
  Product : Product  OutDataTypeStr=fixdt(1,32,30)  SaturateOnIntegerOverflow=on
  Product1 : Product  OutDataTypeStr=fixdt(1,32,30)  SaturateOnIntegerOverflow=on
  Subtract : Sum  Inputs=+-  OutDataTypeStr=fixdt(1,32,30)  SaturateOnIntegerOverflow=on
  Out1 : Outport
  wires:
  In2/1 -> Product/1
  In3/1 -> Product/2
  In1/1 -> Product1/1
  In4/1 -> Product1/2
  Product/1 -> Subtract/1
  Product1/1 -> Subtract/2
  Subtract/1 -> Out1/1

== system HFMA_4B_1_5_9_13/Subsystem/HFMA13/Covariance Matrix/R21/Leaky Average ==
  p[n] : Inport
  RESET : Inport  Port=2
  Add : Sum  OutDataTypeStr=fixdt(1,32,30)  SaturateOnIntegerOverflow=on
  Delay : Delay  DelayLength=1  ExternalReset=Level
      settings: InputPortMap=u0,r5
  Gain : Gain  Gain=2^-k_avg  OutDataTypeStr=fixdt(1,32,30)  SaturateOnIntegerOverflow=on
  Minus : Sum  Inputs=+-  OutDataTypeStr=fixdt(1,32,30)  SaturateOnIntegerOverflow=on
  Rij Out : Outport
  wires:
  p[n]/1 -> Minus/1
  Minus/1 -> Gain/1
  Gain/1 -> Add/1
  Add/1 -> Delay/1
  Delay/1 -> Rij Out/1, Minus/2, Add/2
  RESET/1 -> Delay/2

== system HFMA_4B_1_5_9_13/Subsystem/HFMA13/Covariance Matrix/R21/Leaky Average1 ==
  p[n] : Inport
  RESET : Inport  Port=2
  Add : Sum  OutDataTypeStr=fixdt(1,32,30)  SaturateOnIntegerOverflow=on
  Delay : Delay  DelayLength=1  ExternalReset=Level
      settings: InputPortMap=u0,r5
  Gain : Gain  Gain=2^-k_avg  OutDataTypeStr=fixdt(1,32,30)  SaturateOnIntegerOverflow=on
  Minus : Sum  Inputs=+-  OutDataTypeStr=fixdt(1,32,30)  SaturateOnIntegerOverflow=on
  Rij Out : Outport
  wires:
  p[n]/1 -> Minus/1
  Minus/1 -> Gain/1
  Gain/1 -> Add/1
  Add/1 -> Delay/1
  Delay/1 -> Rij Out/1, Minus/2, Add/2
  RESET/1 -> Delay/2

== system HFMA_4B_1_5_9_13/Subsystem/HFMA13/Covariance Matrix/R21/ac_bd ==
  In1 : Inport
  In2 : Inport  Port=2
  In3 : Inport  Port=3
  In4 : Inport  Port=4
  Add : Sum  OutDataTypeStr=fixdt(1,32,30)  SaturateOnIntegerOverflow=on
  Product : Product  OutDataTypeStr=fixdt(1,32,30)  SaturateOnIntegerOverflow=on
  Product1 : Product  OutDataTypeStr=fixdt(1,32,30)  SaturateOnIntegerOverflow=on
  Out1 : Outport
  wires:
  In1/1 -> Product/1
  In3/1 -> Product/2
  In2/1 -> Product1/1
  In4/1 -> Product1/2
  Product/1 -> Add/1
  Product1/1 -> Add/2
  Add/1 -> Out1/1

== system HFMA_4B_1_5_9_13/Subsystem/HFMA13/Covariance Matrix/R21/bc_ad ==
  In1 : Inport
  In2 : Inport  Port=2
  In3 : Inport  Port=3
  In4 : Inport  Port=4
  Product : Product  OutDataTypeStr=fixdt(1,32,30)  SaturateOnIntegerOverflow=on
  Product1 : Product  OutDataTypeStr=fixdt(1,32,30)  SaturateOnIntegerOverflow=on
  Subtract : Sum  Inputs=+-  OutDataTypeStr=fixdt(1,32,30)  SaturateOnIntegerOverflow=on
  Out1 : Outport
  wires:
  In2/1 -> Product/1
  In3/1 -> Product/2
  In1/1 -> Product1/1
  In4/1 -> Product1/2
  Product/1 -> Subtract/1
  Product1/1 -> Subtract/2
  Subtract/1 -> Out1/1

== system HFMA_4B_1_5_9_13/Subsystem/HFMA5/Covariance Matrix/R1/Leaky Average ==
  p[n] : Inport
  RESET : Inport  Port=2
  Add : Sum  OutDataTypeStr=fixdt(1,32,30)  SaturateOnIntegerOverflow=on
  Delay : Delay  DelayLength=1  ExternalReset=Level
      settings: InputPortMap=u0,r5
  Gain : Gain  Gain=2^-k_avg  OutDataTypeStr=fixdt(1,32,30)  SaturateOnIntegerOverflow=on
  Minus : Sum  Inputs=+-  OutDataTypeStr=fixdt(1,32,30)  SaturateOnIntegerOverflow=on
  Rij Out : Outport
  wires:
  p[n]/1 -> Minus/1
  Minus/1 -> Gain/1
  Gain/1 -> Add/1
  Add/1 -> Delay/1
  Delay/1 -> Rij Out/1, Minus/2, Add/2
  RESET/1 -> Delay/2

== system HFMA_4B_1_5_9_13/Subsystem/HFMA5/Covariance Matrix/R1/Leaky Average1 ==
  p[n] : Inport
  RESET : Inport  Port=2
  Add : Sum  OutDataTypeStr=fixdt(1,32,30)  SaturateOnIntegerOverflow=on
  Delay : Delay  DelayLength=1  ExternalReset=Level
      settings: InputPortMap=u0,r5
  Gain : Gain  Gain=2^-k_avg  OutDataTypeStr=fixdt(1,32,30)  SaturateOnIntegerOverflow=on
  Minus : Sum  Inputs=+-  OutDataTypeStr=fixdt(1,32,30)  SaturateOnIntegerOverflow=on
  Rij Out : Outport
  wires:
  p[n]/1 -> Minus/1
  Minus/1 -> Gain/1
  Gain/1 -> Add/1
  Add/1 -> Delay/1
  Delay/1 -> Rij Out/1, Minus/2, Add/2
  RESET/1 -> Delay/2

== system HFMA_4B_1_5_9_13/Subsystem/HFMA5/Covariance Matrix/R1/ac_bd ==
  In1 : Inport
  In2 : Inport  Port=2
  In3 : Inport  Port=3
  In4 : Inport  Port=4
  Add : Sum  OutDataTypeStr=fixdt(1,32,30)  SaturateOnIntegerOverflow=on
  Product : Product  OutDataTypeStr=fixdt(1,32,30)  SaturateOnIntegerOverflow=on
  Product1 : Product  OutDataTypeStr=fixdt(1,32,30)  SaturateOnIntegerOverflow=on
  Out1 : Outport
  wires:
  In1/1 -> Product/1
  In3/1 -> Product/2
  In2/1 -> Product1/1
  In4/1 -> Product1/2
  Product/1 -> Add/1
  Product1/1 -> Add/2
  Add/1 -> Out1/1

== system HFMA_4B_1_5_9_13/Subsystem/HFMA5/Covariance Matrix/R1/bc_ad ==
  In1 : Inport
  In2 : Inport  Port=2
  In3 : Inport  Port=3
  In4 : Inport  Port=4
  Product : Product  OutDataTypeStr=fixdt(1,32,30)  SaturateOnIntegerOverflow=on
  Product1 : Product  OutDataTypeStr=fixdt(1,32,30)  SaturateOnIntegerOverflow=on
  Subtract : Sum  Inputs=+-  OutDataTypeStr=fixdt(1,32,30)  SaturateOnIntegerOverflow=on
  Out1 : Outport
  wires:
  In2/1 -> Product/1
  In3/1 -> Product/2
  In1/1 -> Product1/1
  In4/1 -> Product1/2
  Product/1 -> Subtract/1
  Product1/1 -> Subtract/2
  Subtract/1 -> Out1/1

== system HFMA_4B_1_5_9_13/Subsystem/HFMA5/Covariance Matrix/R2/Leaky Average ==
  p[n] : Inport
  RESET : Inport  Port=2
  Add : Sum  OutDataTypeStr=fixdt(1,32,30)  SaturateOnIntegerOverflow=on
  Delay : Delay  DelayLength=1  ExternalReset=Level
      settings: InputPortMap=u0,r5
  Gain : Gain  Gain=2^-k_avg  OutDataTypeStr=fixdt(1,32,30)  SaturateOnIntegerOverflow=on
  Minus : Sum  Inputs=+-  OutDataTypeStr=fixdt(1,32,30)  SaturateOnIntegerOverflow=on
  Rij Out : Outport
  wires:
  p[n]/1 -> Minus/1
  Minus/1 -> Gain/1
  Gain/1 -> Add/1
  Add/1 -> Delay/1
  Delay/1 -> Rij Out/1, Minus/2, Add/2
  RESET/1 -> Delay/2

== system HFMA_4B_1_5_9_13/Subsystem/HFMA5/Covariance Matrix/R2/Leaky Average1 ==
  p[n] : Inport
  RESET : Inport  Port=2
  Add : Sum  OutDataTypeStr=fixdt(1,32,30)  SaturateOnIntegerOverflow=on
  Delay : Delay  DelayLength=1  ExternalReset=Level
      settings: InputPortMap=u0,r5
  Gain : Gain  Gain=2^-k_avg  OutDataTypeStr=fixdt(1,32,30)  SaturateOnIntegerOverflow=on
  Minus : Sum  Inputs=+-  OutDataTypeStr=fixdt(1,32,30)  SaturateOnIntegerOverflow=on
  Rij Out : Outport
  wires:
  p[n]/1 -> Minus/1
  Minus/1 -> Gain/1
  Gain/1 -> Add/1
  Add/1 -> Delay/1
  Delay/1 -> Rij Out/1, Minus/2, Add/2
  RESET/1 -> Delay/2

== system HFMA_4B_1_5_9_13/Subsystem/HFMA5/Covariance Matrix/R2/ac_bd ==
  In1 : Inport
  In2 : Inport  Port=2
  In3 : Inport  Port=3
  In4 : Inport  Port=4
  Add : Sum  OutDataTypeStr=fixdt(1,32,30)  SaturateOnIntegerOverflow=on
  Product : Product  OutDataTypeStr=fixdt(1,32,30)  SaturateOnIntegerOverflow=on
  Product1 : Product  OutDataTypeStr=fixdt(1,32,30)  SaturateOnIntegerOverflow=on
  Out1 : Outport
  wires:
  In1/1 -> Product/1
  In3/1 -> Product/2
  In2/1 -> Product1/1
  In4/1 -> Product1/2
  Product/1 -> Add/1
  Product1/1 -> Add/2
  Add/1 -> Out1/1

== system HFMA_4B_1_5_9_13/Subsystem/HFMA5/Covariance Matrix/R2/bc_ad ==
  In1 : Inport
  In2 : Inport  Port=2
  In3 : Inport  Port=3
  In4 : Inport  Port=4
  Product : Product  OutDataTypeStr=fixdt(1,32,30)  SaturateOnIntegerOverflow=on
  Product1 : Product  OutDataTypeStr=fixdt(1,32,30)  SaturateOnIntegerOverflow=on
  Subtract : Sum  Inputs=+-  OutDataTypeStr=fixdt(1,32,30)  SaturateOnIntegerOverflow=on
  Out1 : Outport
  wires:
  In2/1 -> Product/1
  In3/1 -> Product/2
  In1/1 -> Product1/1
  In4/1 -> Product1/2
  Product/1 -> Subtract/1
  Product1/1 -> Subtract/2
  Subtract/1 -> Out1/1

== system HFMA_4B_1_5_9_13/Subsystem/HFMA5/Covariance Matrix/R21/Leaky Average ==
  p[n] : Inport
  RESET : Inport  Port=2
  Add : Sum  OutDataTypeStr=fixdt(1,32,30)  SaturateOnIntegerOverflow=on
  Delay : Delay  DelayLength=1  ExternalReset=Level
      settings: InputPortMap=u0,r5
  Gain : Gain  Gain=2^-k_avg  OutDataTypeStr=fixdt(1,32,30)  SaturateOnIntegerOverflow=on
  Minus : Sum  Inputs=+-  OutDataTypeStr=fixdt(1,32,30)  SaturateOnIntegerOverflow=on
  Rij Out : Outport
  wires:
  p[n]/1 -> Minus/1
  Minus/1 -> Gain/1
  Gain/1 -> Add/1
  Add/1 -> Delay/1
  Delay/1 -> Rij Out/1, Minus/2, Add/2
  RESET/1 -> Delay/2

== system HFMA_4B_1_5_9_13/Subsystem/HFMA5/Covariance Matrix/R21/Leaky Average1 ==
  p[n] : Inport
  RESET : Inport  Port=2
  Add : Sum  OutDataTypeStr=fixdt(1,32,30)  SaturateOnIntegerOverflow=on
  Delay : Delay  DelayLength=1  ExternalReset=Level
      settings: InputPortMap=u0,r5
  Gain : Gain  Gain=2^-k_avg  OutDataTypeStr=fixdt(1,32,30)  SaturateOnIntegerOverflow=on
  Minus : Sum  Inputs=+-  OutDataTypeStr=fixdt(1,32,30)  SaturateOnIntegerOverflow=on
  Rij Out : Outport
  wires:
  p[n]/1 -> Minus/1
  Minus/1 -> Gain/1
  Gain/1 -> Add/1
  Add/1 -> Delay/1
  Delay/1 -> Rij Out/1, Minus/2, Add/2
  RESET/1 -> Delay/2

== system HFMA_4B_1_5_9_13/Subsystem/HFMA5/Covariance Matrix/R21/ac_bd ==
  In1 : Inport
  In2 : Inport  Port=2
  In3 : Inport  Port=3
  In4 : Inport  Port=4
  Add : Sum  OutDataTypeStr=fixdt(1,32,30)  SaturateOnIntegerOverflow=on
  Product : Product  OutDataTypeStr=fixdt(1,32,30)  SaturateOnIntegerOverflow=on
  Product1 : Product  OutDataTypeStr=fixdt(1,32,30)  SaturateOnIntegerOverflow=on
  Out1 : Outport
  wires:
  In1/1 -> Product/1
  In3/1 -> Product/2
  In2/1 -> Product1/1
  In4/1 -> Product1/2
  Product/1 -> Add/1
  Product1/1 -> Add/2
  Add/1 -> Out1/1

== system HFMA_4B_1_5_9_13/Subsystem/HFMA5/Covariance Matrix/R21/bc_ad ==
  In1 : Inport
  In2 : Inport  Port=2
  In3 : Inport  Port=3
  In4 : Inport  Port=4
  Product : Product  OutDataTypeStr=fixdt(1,32,30)  SaturateOnIntegerOverflow=on
  Product1 : Product  OutDataTypeStr=fixdt(1,32,30)  SaturateOnIntegerOverflow=on
  Subtract : Sum  Inputs=+-  OutDataTypeStr=fixdt(1,32,30)  SaturateOnIntegerOverflow=on
  Out1 : Outport
  wires:
  In2/1 -> Product/1
  In3/1 -> Product/2
  In1/1 -> Product1/1
  In4/1 -> Product1/2
  Product/1 -> Subtract/1
  Product1/1 -> Subtract/2
  Subtract/1 -> Out1/1

== system HFMA_4B_1_5_9_13/Subsystem/HFMA9/Covariance Matrix/R1/Leaky Average ==
  p[n] : Inport
  RESET : Inport  Port=2
  Add : Sum  OutDataTypeStr=fixdt(1,32,30)  SaturateOnIntegerOverflow=on
  Delay : Delay  DelayLength=1  ExternalReset=Level
      settings: InputPortMap=u0,r5
  Gain : Gain  Gain=2^-k_avg  OutDataTypeStr=fixdt(1,32,30)  SaturateOnIntegerOverflow=on
  Minus : Sum  Inputs=+-  OutDataTypeStr=fixdt(1,32,30)  SaturateOnIntegerOverflow=on
  Rij Out : Outport
  wires:
  p[n]/1 -> Minus/1
  Minus/1 -> Gain/1
  Gain/1 -> Add/1
  Add/1 -> Delay/1
  Delay/1 -> Rij Out/1, Minus/2, Add/2
  RESET/1 -> Delay/2

== system HFMA_4B_1_5_9_13/Subsystem/HFMA9/Covariance Matrix/R1/Leaky Average1 ==
  p[n] : Inport
  RESET : Inport  Port=2
  Add : Sum  OutDataTypeStr=fixdt(1,32,30)  SaturateOnIntegerOverflow=on
  Delay : Delay  DelayLength=1  ExternalReset=Level
      settings: InputPortMap=u0,r5
  Gain : Gain  Gain=2^-k_avg  OutDataTypeStr=fixdt(1,32,30)  SaturateOnIntegerOverflow=on
  Minus : Sum  Inputs=+-  OutDataTypeStr=fixdt(1,32,30)  SaturateOnIntegerOverflow=on
  Rij Out : Outport
  wires:
  p[n]/1 -> Minus/1
  Minus/1 -> Gain/1
  Gain/1 -> Add/1
  Add/1 -> Delay/1
  Delay/1 -> Rij Out/1, Minus/2, Add/2
  RESET/1 -> Delay/2

== system HFMA_4B_1_5_9_13/Subsystem/HFMA9/Covariance Matrix/R1/ac_bd ==
  In1 : Inport
  In2 : Inport  Port=2
  In3 : Inport  Port=3
  In4 : Inport  Port=4
  Add : Sum  OutDataTypeStr=fixdt(1,32,30)  SaturateOnIntegerOverflow=on
  Product : Product  OutDataTypeStr=fixdt(1,32,30)  SaturateOnIntegerOverflow=on
  Product1 : Product  OutDataTypeStr=fixdt(1,32,30)  SaturateOnIntegerOverflow=on
  Out1 : Outport
  wires:
  In1/1 -> Product/1
  In3/1 -> Product/2
  In2/1 -> Product1/1
  In4/1 -> Product1/2
  Product/1 -> Add/1
  Product1/1 -> Add/2
  Add/1 -> Out1/1

== system HFMA_4B_1_5_9_13/Subsystem/HFMA9/Covariance Matrix/R1/bc_ad ==
  In1 : Inport
  In2 : Inport  Port=2
  In3 : Inport  Port=3
  In4 : Inport  Port=4
  Product : Product  OutDataTypeStr=fixdt(1,32,30)  SaturateOnIntegerOverflow=on
  Product1 : Product  OutDataTypeStr=fixdt(1,32,30)  SaturateOnIntegerOverflow=on
  Subtract : Sum  Inputs=+-  OutDataTypeStr=fixdt(1,32,30)  SaturateOnIntegerOverflow=on
  Out1 : Outport
  wires:
  In2/1 -> Product/1
  In3/1 -> Product/2
  In1/1 -> Product1/1
  In4/1 -> Product1/2
  Product/1 -> Subtract/1
  Product1/1 -> Subtract/2
  Subtract/1 -> Out1/1

== system HFMA_4B_1_5_9_13/Subsystem/HFMA9/Covariance Matrix/R2/Leaky Average ==
  p[n] : Inport
  RESET : Inport  Port=2
  Add : Sum  OutDataTypeStr=fixdt(1,32,30)  SaturateOnIntegerOverflow=on
  Delay : Delay  DelayLength=1  ExternalReset=Level
      settings: InputPortMap=u0,r5
  Gain : Gain  Gain=2^-k_avg  OutDataTypeStr=fixdt(1,32,30)  SaturateOnIntegerOverflow=on
  Minus : Sum  Inputs=+-  OutDataTypeStr=fixdt(1,32,30)  SaturateOnIntegerOverflow=on
  Rij Out : Outport
  wires:
  p[n]/1 -> Minus/1
  Minus/1 -> Gain/1
  Gain/1 -> Add/1
  Add/1 -> Delay/1
  Delay/1 -> Rij Out/1, Minus/2, Add/2
  RESET/1 -> Delay/2

== system HFMA_4B_1_5_9_13/Subsystem/HFMA9/Covariance Matrix/R2/Leaky Average1 ==
  p[n] : Inport
  RESET : Inport  Port=2
  Add : Sum  OutDataTypeStr=fixdt(1,32,30)  SaturateOnIntegerOverflow=on
  Delay : Delay  DelayLength=1  ExternalReset=Level
      settings: InputPortMap=u0,r5
  Gain : Gain  Gain=2^-k_avg  OutDataTypeStr=fixdt(1,32,30)  SaturateOnIntegerOverflow=on
  Minus : Sum  Inputs=+-  OutDataTypeStr=fixdt(1,32,30)  SaturateOnIntegerOverflow=on
  Rij Out : Outport
  wires:
  p[n]/1 -> Minus/1
  Minus/1 -> Gain/1
  Gain/1 -> Add/1
  Add/1 -> Delay/1
  Delay/1 -> Rij Out/1, Minus/2, Add/2
  RESET/1 -> Delay/2

== system HFMA_4B_1_5_9_13/Subsystem/HFMA9/Covariance Matrix/R2/ac_bd ==
  In1 : Inport
  In2 : Inport  Port=2
  In3 : Inport  Port=3
  In4 : Inport  Port=4
  Add : Sum  OutDataTypeStr=fixdt(1,32,30)  SaturateOnIntegerOverflow=on
  Product : Product  OutDataTypeStr=fixdt(1,32,30)  SaturateOnIntegerOverflow=on
  Product1 : Product  OutDataTypeStr=fixdt(1,32,30)  SaturateOnIntegerOverflow=on
  Out1 : Outport
  wires:
  In1/1 -> Product/1
  In3/1 -> Product/2
  In2/1 -> Product1/1
  In4/1 -> Product1/2
  Product/1 -> Add/1
  Product1/1 -> Add/2
  Add/1 -> Out1/1

== system HFMA_4B_1_5_9_13/Subsystem/HFMA9/Covariance Matrix/R2/bc_ad ==
  In1 : Inport
  In2 : Inport  Port=2
  In3 : Inport  Port=3
  In4 : Inport  Port=4
  Product : Product  OutDataTypeStr=fixdt(1,32,30)  SaturateOnIntegerOverflow=on
  Product1 : Product  OutDataTypeStr=fixdt(1,32,30)  SaturateOnIntegerOverflow=on
  Subtract : Sum  Inputs=+-  OutDataTypeStr=fixdt(1,32,30)  SaturateOnIntegerOverflow=on
  Out1 : Outport
  wires:
  In2/1 -> Product/1
  In3/1 -> Product/2
  In1/1 -> Product1/1
  In4/1 -> Product1/2
  Product/1 -> Subtract/1
  Product1/1 -> Subtract/2
  Subtract/1 -> Out1/1

== system HFMA_4B_1_5_9_13/Subsystem/HFMA9/Covariance Matrix/R21/Leaky Average ==
  p[n] : Inport
  RESET : Inport  Port=2
  Add : Sum  OutDataTypeStr=fixdt(1,32,30)  SaturateOnIntegerOverflow=on
  Delay : Delay  DelayLength=1  ExternalReset=Level
      settings: InputPortMap=u0,r5
  Gain : Gain  Gain=2^-k_avg  OutDataTypeStr=fixdt(1,32,30)  SaturateOnIntegerOverflow=on
  Minus : Sum  Inputs=+-  OutDataTypeStr=fixdt(1,32,30)  SaturateOnIntegerOverflow=on
  Rij Out : Outport
  wires:
  p[n]/1 -> Minus/1
  Minus/1 -> Gain/1
  Gain/1 -> Add/1
  Add/1 -> Delay/1
  Delay/1 -> Rij Out/1, Minus/2, Add/2
  RESET/1 -> Delay/2

== system HFMA_4B_1_5_9_13/Subsystem/HFMA9/Covariance Matrix/R21/Leaky Average1 ==
  p[n] : Inport
  RESET : Inport  Port=2
  Add : Sum  OutDataTypeStr=fixdt(1,32,30)  SaturateOnIntegerOverflow=on
  Delay : Delay  DelayLength=1  ExternalReset=Level
      settings: InputPortMap=u0,r5
  Gain : Gain  Gain=2^-k_avg  OutDataTypeStr=fixdt(1,32,30)  SaturateOnIntegerOverflow=on
  Minus : Sum  Inputs=+-  OutDataTypeStr=fixdt(1,32,30)  SaturateOnIntegerOverflow=on
  Rij Out : Outport
  wires:
  p[n]/1 -> Minus/1
  Minus/1 -> Gain/1
  Gain/1 -> Add/1
  Add/1 -> Delay/1
  Delay/1 -> Rij Out/1, Minus/2, Add/2
  RESET/1 -> Delay/2
